simulink model "testGNModel"  (R2025b)
settings: Solver=FixedStepAuto  StartTime=0.0  StopTime=30  FixedStep=Ts  RelTol=1e-3
PreLoadFcn:
  | init_model;
values from neighbouring files (symbols this model uses):
  acceptance_radius = 0.5    [init_model.m]
  cruise_speed = 2.0    (= 2)    [init_model.m]
  gps_noise_variance = 0.05    [init_model.m]
  tau_delay = 0.2    [init_model.m]
  Ts = 0.01    [init_model.m]
  waypoints = [  0,   0,   0 ... (first row only)    [init_model.m]
libraries: uavutilslib x1
settings Model: Creator=carte  LastModifiedBy=carte

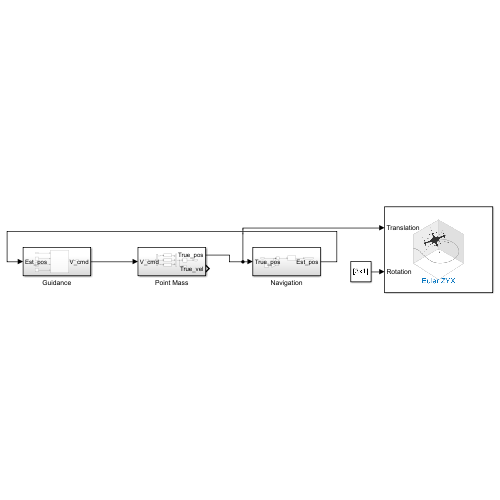
[thumbnail: Simulink's stored preview of the top-level diagram]
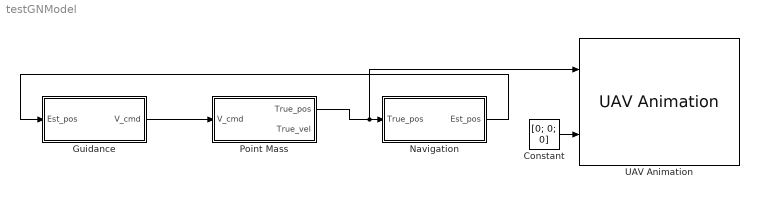
== system testGNModel ==
  Constant : Constant  Value=[0; 0; 0]
  Guidance : Subsystem
  Navigation : Subsystem
  Point Mass : Subsystem
  UAV Animation : uavutilslib/UAV Animation  NumUAV=1  DynamicUAVConfig=off  UAVType=Multirotor  UAVSize=1  UAVColor=[1 0 0]  UAVTrajectoryAlpha=1  InertialZDirection=Down  RotationFormat=Euler ZYX  DrawMarkers=off  SampleTime=Ts
  wires:
  Guidance/1(V_cmd) -> Point Mass/1(V_cmd)
  Point Mass/1(True_pos) -> UAV Animation/1, Navigation/1(True_pos)
  Navigation/1(Est_pos) -> Guidance/1(Est_pos)
  Constant/1 -> UAV Animation/2

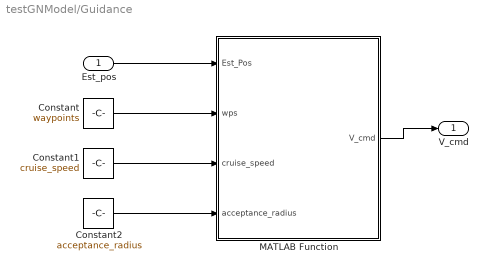
== system testGNModel/Guidance ==
  Est_pos : Inport  PortDimensions=3
  Constant : Constant  Value=waypoints
  Constant1 : Constant  Value=cruise_speed
  Constant2 : Constant  Value=acceptance_radius
  MATLAB Function : MATLAB Function  TreatAsAtomicUnit=on
  V_cmd : Outport
  wires:
  Est_pos/1 -> MATLAB Function/1(Est_Pos)
  MATLAB Function/1(V_cmd) -> V_cmd/1
  Constant/1 -> MATLAB Function/2(wps)
  Constant1/1 -> MATLAB Function/3(cruise_speed)
  Constant2/1 -> MATLAB Function/4(acceptance_radius)

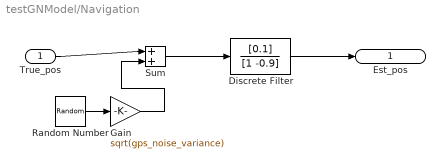
== system testGNModel/Navigation ==
  True_pos : Inport  PortDimensions=3
  Discrete Filter : DiscreteFilter  Numerator=[0.1]  Denominator=[1 -0.9]
  Gain : Gain  Gain=sqrt(gps_noise_variance)
  Random Number : RandomNumber  Mean=[0; 0; 0]  Variance=[1; 1; 1]  SampleTime=Ts
  Sum : Sum  Inputs=|++
  Est_pos : Outport  PortDimensions=3
  wires:
  True_pos/1 -> Sum/1
  Random Number/1 -> Gain/1
  Gain/1 -> Sum/2
  Sum/1 -> Discrete Filter/1
  Discrete Filter/1 -> Est_pos/1

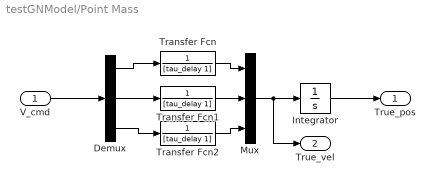
== system testGNModel/Point Mass ==
  V_cmd : Inport
  Demux : Demux  Outputs=3
  Integrator : Integrator
  Mux : Mux  Inputs=3
  Transfer Fcn : TransferFcn  Denominator=[tau_delay 1]
  Transfer Fcn1 : TransferFcn  Denominator=[tau_delay 1]
  Transfer Fcn2 : TransferFcn  Denominator=[tau_delay 1]
  True_pos : Outport
  True_vel : Outport  Port=2
  wires:
  Integrator/1 -> True_pos/1
  V_cmd/1 -> Demux/1
  Demux/1 -> Transfer Fcn/1
  Demux/2 -> Transfer Fcn1/1
  Demux/3 -> Transfer Fcn2/1
  Transfer Fcn1/1 -> Mux/2
  Transfer Fcn/1 -> Mux/1
  Transfer Fcn2/1 -> Mux/3
  Mux/1 -> True_vel/1, Integrator/1

== matlab function testGNModel/Guidance/MATLAB Function ==
  data: Est_Pos input; V_cmd output; wps input; cruise_speed input; acceptance_radius input
function V_cmd = multirotor_guidance(Est_Pos, wps, cruise_speed, acceptance_radius)
    % Declare a persistent variable to keep track of the active waypoint index
    persistent wp_idx;
    if isempty(wp_idx)
        wp_idx = 1; 
    end
    
    % 1. Safety Check: If we have completed all waypoints, hold position (zero velocity)
    if wp_idx > size(wps, 1)
        V_cmd = [0; 0; 0];
        return;
    end
    
    % 2. Extract current target waypoint position (must be a 3x1 column vector)
    target = wps(wp_idx, : )';
    
    % 3. Calculate distance and directional vector to the target
    direction = target - Est_Pos;
    distance = norm(direction);
    
    % 4. Waypoint Switching Logic
    % If we enter the acceptance sphere, advance to the next target waypoint
    if distance < acceptance_radius
        wp_idx = wp_idx + 1;
    end
    
    % 5. Generate Velocity Output
    if distance > 0.01
        % Normalize direction to a unit vector and scale by cruise speed
        V_cmd = (direction / distance) * cruise_speed;
    else
        V_cmd = [0; 0; 0];
    end
end
